simulink model "Hinf_linear_sim"  (R2026a)
settings: Solver=VariableStepAuto
undefined symbols (not defined in the file): A, Ak, B, Bk, Ck, Cq, Dk
settings Model: Creator=rebec  LastModifiedBy=rebec

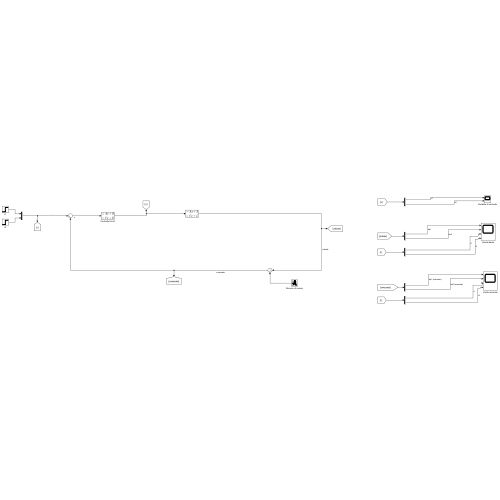
[thumbnail: Simulink's stored preview of the top-level diagram]
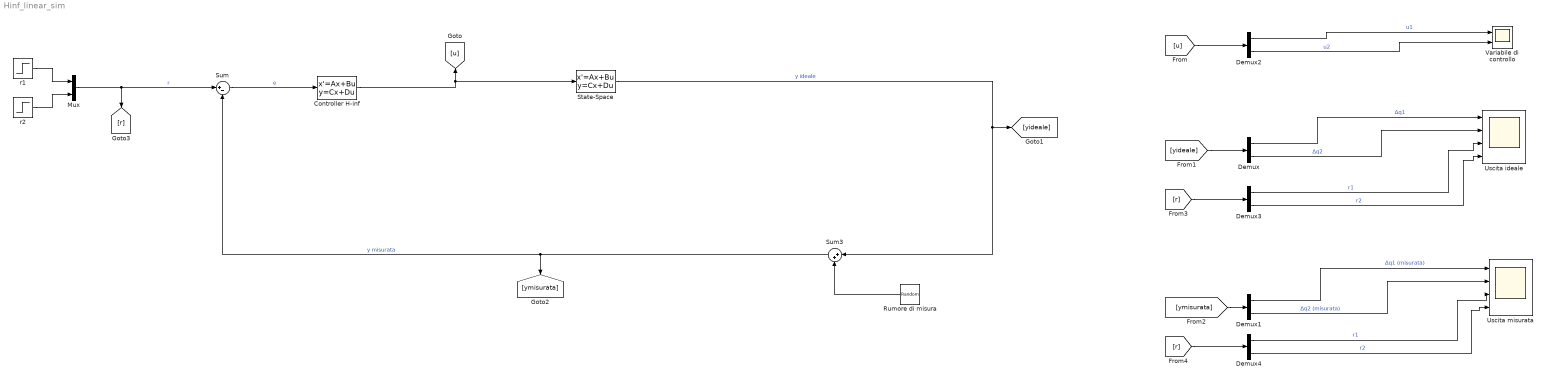
== system Hinf_linear_sim ==
  Controller H-inf : StateSpace  A=Ak  B=Bk  C=Ck  D=Dk  InitialCondition=0
  Demux{,1..4} (5 alike) : Demux  Outputs=2
  Mux : Mux  Inputs=2
  Rumore di misura : RandomNumber  Variance=(0.05*pi/180)^2  Seed=20260826  SampleTime=0.002
  State-Space : StateSpace  A=A  B=B  C=Cq  D=zeros(2,2);  InitialCondition=0
  Sum : Sum  Inputs=|+-
  Sum3 : Sum  Inputs=|++
  Uscita ideale : Scope  NumInputPorts=4
      settings: Title=y (uscita ideale)  ActiveDisplayYMinimum=-0.6065472521807  ActiveDisplayYMaximum=0.64249935531189384
  Uscita misurata : Scope  NumInputPorts=4
      settings: Title=y (uscita ideale)  ActiveDisplayYMinimum=-0.54348624607883766  ActiveDisplayYMaximum=0.4563878411340912
  Variabile di controllo : Scope  NumInputPorts=2
      settings: ActiveDisplayYMinimum=-2.6959450601265313  ActiveDisplayYMaximum=5.9059369724787079  DataLoggingVariableName=ScopeData2
  r1 : Step  FinalValue=5*pi/180  SampleTime=0
  r2 : Step  FinalValue=0  SampleTime=0
  wires:
  State-Space/1 -> [yideale], Sum3/1  "y ideale"
  r2/1 -> Mux/2
  Sum/1 -> Controller H-inf/1  "e"
  Rumore di misura/1 -> Sum3/2
  Sum3/1 -> Sum/2, [ymisurata]  "y misurata"
  Mux/1 -> Sum/1, [r]  "r"
  Controller H-inf/1 -> State-Space/1, [u]
  r1/1 -> Mux/1
  Demux4/1 -> Uscita misurata/3  "r1"
  Demux/2 -> Uscita ideale/2  "Δq2"
  Demux3/2 -> Uscita ideale/4  "r2"
  [u] -> Demux2/1
  [yideale] -> Demux/1
  Demux1/1 -> Uscita misurata/1  "Δq1 (misurata)"
  Demux3/1 -> Uscita ideale/3  "r1"
  [ymisurata] -> Demux1/1
  Demux/1 -> Uscita ideale/1  "Δq1"
  Demux1/2 -> Uscita misurata/2  "Δq2 (misurata)"
  Demux2/1 -> Variabile di controllo/1  "u1"
  [r] -> Demux4/1
  Demux2/2 -> Variabile di controllo/2  "u2"
  Demux4/2 -> Uscita misurata/4  "r2"
  [r] -> Demux3/1
